simulink model "testrig_susp_knc"  (R2026a)
settings: Solver=ode23t  StopTime=309  MaxStep=0.05  AbsTol=1e-3  EnableMultiTasking=on
PostLoadFcn:
  | sm_car_load_vehicle_data('none','000');
  | Vehicle = sm_car_vehcfg_setPeopleOnOff(Vehicle,[0 0 0 0 0],'SuspA1');
  | set_param([bdroot '/Axle'],'AxNum','Front');
  | set_param([bdroot '/Axle/Visuals'],'popup_vis_point','Off');
  | 
  | Maneuver = MDatabase.KnC.Sedan_HambaLG;
  | Visual = sm_car_param_visual('default');
undefined symbols (not defined in the file or in its folder): Axle1D, AxleIn, Init, RaceFix, RaceSpin, X, Y, Z
libraries: sm_lib x9, sm_car_testrig_utilities_lib x6, fl_lib x4, Damper_Element x2, Spring_Element x2, nesl_utility x1, Damper_Control x1, Suspension x1, World_Config_Utilities x1
CloseFcn:
  | clear simlog_sm_car_testrig_quarter_car
  | clear logsout_sm_car_testrig_quarter_car
Description:
  | Half Car Testrig, Pullrod
  | 
  | Copyright 2021-2026 The MathWorks, Inc.
settings Model: Creator=smiller  LastModifiedBy=smiller
settings DataIOCC: SignalLoggingName=logsout_sm_car_testrig_quarter_car
settings SimscapeCC: SimscapeNominalValues="[{\"value\":\"1\",\"unit\":\"A\"},{\"value\":\"1\",\"unit\":\"bar\"},{\"value\":\"1\",\"unit\":\"cm^2\"},{\"value\":\"1\",\"unit\":\"cm^3/s\"},{\"value\":\"1\",\"unit\":\"kJ/kg\"},{\"value\":\"1\",\"unit\":\"kW\"},{\"value\":\"1\",\"unit\":\"l\"},{\"value\":\"1\",\"unit\":\"N\"},{\"value\":\"1\",\"unit\":\"N*m\"},{\"value\":\"1\",\"unit\":\"V\"}]"  SimscapeLogSimulationStatistics=on  SimscapeLogName=simlog_sm_car_testrig_quarter_car  SimscapeLogLimitData=off  SimscapeOperatingPoint=op
settings DiagnosticsConfigSet: SimMechanicsUnconnectedFramePorts=none  SimMechanicsConflictingReferenceFrames=none
settings ExplorerConfigSet: InternalSimMechanicsExplorerSettings="<ExplorerConfiguration><canonicalview>default</canonicalview><AnimationSetting><BasePlaybackSpeed>1.0</BasePlaybackSpeed><PlaybackSpeedFactor>16.0</PlaybackSpeedFactor></AnimationSetting><TilePanel><TileInfo><Tiles Columns=\"1\" Count=\"1\" Rows=\"1\"><Column Weight=\"1\"/><Row Weight=\"1\"/><Tile Height=\"1\" Width=\"1\" X=\"0\" Y=\"0\"/></Tiles></TileInfo><SceneInfo><SceneViewer><BGColor><R>1</R><G>1</G><B>1</B></BGColor><Camera><DoPerspective>off</DoPerspective><Position><X>0.571928528858414942</X><Y>-0.579111562749420217</Y><Z>0.83606068842340453</Z></Position><Center><X>-0.00542174033121090027</X><Y>-0.00176129355979437463</Y><Z>0.258710419233778688</Z></Center><Up><X>-0.408248290463863073</X><Y>0.408248290463863073</Y><Z>0.816496580927726145</Z></Up><ViewLimDist>1</ViewLimDist><YLim>0.718679582981457732</YLim><XLim>0.891323281686500546</XLim></Camera></SceneViewer></SceneInfo></TilePanel><MechEditorPanel><Cameras/><GfxPanelCameraMap/><VideoCreator><PlaybackSpeedRatio>1.0</PlaybackSpeedRatio><FrameRate>30</FrameRate><VideoFormat>Motion JPEG AVI</VideoFormat><FrameSize>auto</FrameSize></VideoCreator></MechEditorPanel></ExplorerConfiguration>"

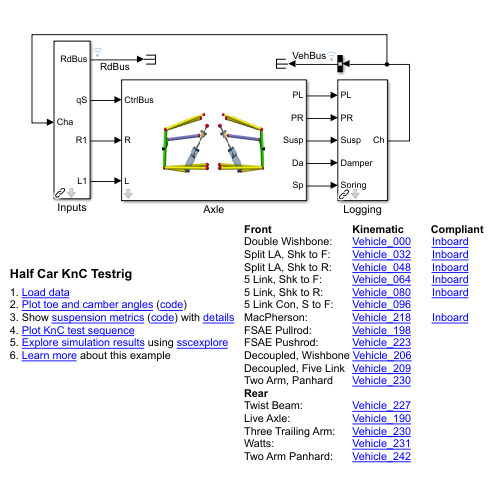
[thumbnail: Simulink's stored preview of the top-level diagram]
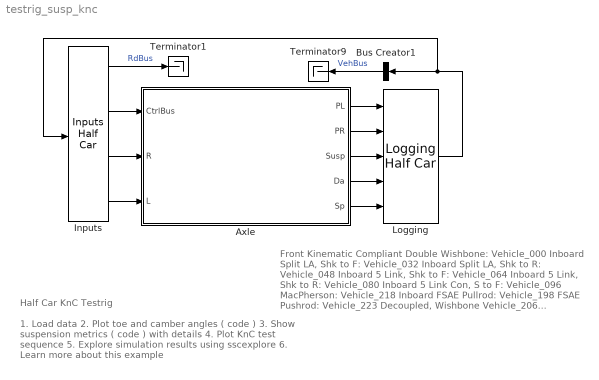
== system testrig_susp_knc ==
  note: Half Car KnC Testrig
  note: 1. Load data
      | 2. Plot toe and camber angles ( code )
      | 3. Show suspension metrics ( code ) with details
      | 4. Plot KnC test sequence
      | 5. Explore simulation results using sscexplore
      | 6. Learn more about this example
  note: Front Kinematic Compliant
      | Double Wishbone: Vehicle_000 Inboard
      | Split LA, Shk to F: Vehicle_032 Inboard
      | Split LA, Shk to R: Vehicle_048 Inboard
      | 5 Link, Shk to F: Vehicle_064 Inboard
      | 5 Link, Shk to R: Vehicle_080 Inboard
      | 5 Link Con, S to F: Vehicle_096
      | MacPherson: Vehicle_218 Inboard
      | FSAE Pullrod: Vehicle_198
      | FSAE Pushrod: Vehicle_223
      | Decoupled, Wishbone Vehicle_206
      | Decoupled, Five Link Vehicle_209
      | Two Arm, Panhard Vehicle_230
      | Rear
      | Twist Beam: Vehicle_227
      | Live Axle: Vehicle_190
      | Three Trailing Arm: Vehicle_230
      | Watts: Vehicle_231
      | Two Arm Panhard: Vehicle_242
  Axle : Subsystem  mask{AxNum=Front, Vehicle=Vehicle, popup_damper_control=None}
      mask prompts: AxNum "Axle"; Vehicle "Vehicle (structure)"; popup_damper_control "Damper Control"
      mask init:
      | curblk = gcb;
      | 
      | sWctrSet = sm_car_get_sWheelCentre(Vehicle);
      | sWCtr     = sWctrSet(AxNum,:);
      | 
      | tire_radii = sm_car_get_TireRadius(Vehicle);
      | tire_radius = tire_radii(AxNum);
      | 
      | if(AxNum==1)
      |     axleField = 'Axle1';
      |     suspField = 'SuspA1';
      |     tireField = 'TireA1';
      | else
      |     axleField = 'Axle2';
      |     suspField = 'SuspA2';
      |     tireField = 'TireA2';
      | end
      | 
      | if(strcmp(Vehicle.Chassis.(suspField).class.Value,'Decoupled'))
      |     springLparam = Vehicle.Chassis.Spring.(axleField).Heave;
      |     springLclass = Vehicle.Chassis.Spring.(axleField).Heave.class.Value;
      |     springRparam = Vehicle.Chassis.Spring.(axleField).Roll;
      |     springRclass = Vehicle.Chassis.Spring.(axleField).Roll.class.Value;
      |     damperLparam = Vehicle.Chassis.Damper.(axleField).Heave;
      |     damperLclass = Vehicle.Chassis.Damper.(axleField).Heave.class.Value;
      |     damperRparam = Vehicle.Chassis.Damper.(axleField).Roll;
      |     damperRclass = Vehicle.Chassis.Damper.(axleField).Roll.class.Value;
      | elseif(strcmp(Vehicle.Chassis.(suspField).class.Value,'LUT') || ...
      |         strcmp(Vehicle.Chassis.(suspField).class.Value,'Simple') )
      |     springLparam = 0;
      |     springLclass = 'No_Spring';
      |     springRparam = 0;
      |     springRclass = 'No_Spring';
      |     damperLparam = 0;
      |     damperLclass = 'None';
      |     damperRparam = 0;
      |     damperRclass = 'None';
      | elseif(strcmp(Vehicle.Chassis.(suspField).class.Value,'AxleTA2PR') || ...
      |         strcmp(Vehicle.Chassis.(suspField).class.Value,'AxleTA2PRNoSteer') )
      |     springLparam          = Vehicle.Chassis.Spring.(axleField);
      |     springLparam.sTop     = Vehicle.Chassis.Spring.(axleField).sTopL;
      |     springLparam.sBottom  = Vehicle.Chassis.Spring.(axleField).sBottomL;
      |     springLparam.xPreload = Vehicle.Chassis.Spring.(axleField).xPreloadL;
      |     springLparam.fPreload = Vehicle.Chassis.Spring.(axleField).fPreloadL;
      |     springLclass   = strrep(Vehicle.Chassis.Spring.(axleField).class.Value,'Asymmetric','');
      | 
      |     springRparam          = Vehicle.Chassis.Spring.(axleField);
      |     springRparam.sTop     = Vehicle.Chassis.Spring.(axleField).sTopR;
      |     springRparam.sBottom  = Vehicle.Chassis.Spring.(axleField).sBottomR;
      |     springRparam.xPreload = Vehicle.Chassis.Spring.(axleField).xPreloadR;
      |     springRparam.fPreload = Vehicle.Chassis.Spring.(axleField).fPreloadR;
      |     springRclass  =  strrep(Vehicle.Chassis.Spring.(axleField).class.Value,'Asymmetric','');
      |     
      |     damperLparam                 = Vehicle.Chassis.Damper.(axleField);
      |     damperLparam.Damping.sTop    = Vehicle.Chassis.Damper.(axleField).Damping.sTopL;
      |     damperLparam.Damping.sBottom = Vehicle.Chassis.Damper.(axleField).Damping.sBottomL;
      |     damperLclass          = strrep(Vehicle.Chassis.Damper.(axleField).class.Value,'Asymmetric','');
      | 
      |     damperRparam                 = Vehicle.Chassis.Damper.(axleField);
      |     damperRparam.Damping.sTop    = Vehicle.Chassis.Damper.(axleField).Damping.sTopR;
      |     damperRparam.Damping.sBottom = Vehicle.Chassis.Damper.(axleField).Damping.sBottomR;
      |     damperRclass          = strrep(Vehicle.Chassis.Damper.(axleField).class.Value,'Asymmetric','');
      | 
      | else
      |     springLparam = Vehicle.Chassis.Spring.(axleField);
      |     springLclass = Vehicle.Chassis.Spring.(axleField).class.Value;
      |     springRparam = Vehicle.Chassis.Spring.(axleField);
      |     springRclass = Vehicle.Chassis.Spring.(axleField).class.Value;
      |     damperLparam = Vehicle.Chassis.Damper.(axleField);
      |     damperLclass = Vehicle.Chassis.Damper.(axleField).class.Value;
      |     damperRparam = Vehicle.Chassis.Damper.(axleField);
      |     damperRclass = Vehicle.Chassis.Damper.(axleField).class.Value;
      | end
      mask TypeOptions AxNum: Front | Rear
      mask TypeOptions popup_damper_control: Damper Control /popup_damper_control
      mask Display:
      | curblk = gcb;
      | activeVar  = get_param([curblk '/Suspension'],'activevariant');
      | varChoices = get_param([curblk '/Suspension'],'VariantChoices');
      | 
      | varInd = find(strcmp(activeVar,{varChoices(:).Name}));
      | 
      | ActiveVarCmd = get_param(varChoices(varInd).BlockName,'MaskDisplay');
      | eval(ActiveVarCmd);
  Bus Creator1 : BusCreator  Inputs=1
  Inputs : sm_car_testrig_utilities_lib/Inputs Half Car  popup_steering_input=On
  Logging : sm_car_testrig_utilities_lib/Logging Half Car
  Terminator1 : Terminator
  Terminator9 : Terminator
  wires:
  Bus Creator1/1 -> Terminator9/1  "VehBus"
  Logging/1 -> Inputs/1, Bus Creator1/1
  Inputs/1 -> Terminator1/1  "RdBus"
  Inputs/3 -> Axle/2(R)
  Inputs/4 -> Axle/3(L)
  Inputs/2 -> Axle/1("CtrlBus ")
  Axle/1(PL) -> Logging/1
  Axle/2(PR) -> Logging/2
  Axle/3(Susp) -> Logging/3
  Axle/4(" Da") -> Logging/4
  Axle/5(" Sp") -> Logging/5

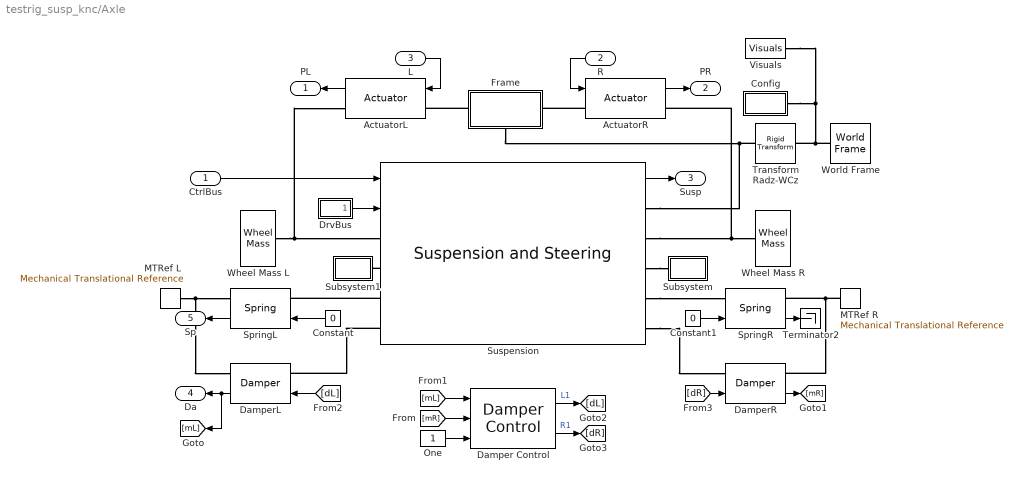
== system testrig_susp_knc/Axle ==
  "CtrlBus " : Inport
  R : Inport  Port=2
  L : Inport  Port=3
  ActuatorL : sm_car_testrig_utilities_lib/Actuator  tire_rad=tire_radius  xCPOffset=Maneuver.xCPOffset
  ActuatorR : sm_car_testrig_utilities_lib/Actuator  tire_rad=tire_radius  xCPOffset=Maneuver.xCPOffset
  Config : Subsystem
  Constant : Constant  Value=0
  Constant1 : Constant  Value=0
  "Damper Control " : Damper_Control/Damper Control   VariantControl=Choice  LabelModeActiveChoice=None  popup_damper_control=None  ControlDamper=Control.Damper.Axle1
      settings: AttributesFormatString=%<popup_damper_control>
  DamperL : Damper_Element/Damper  VariantControl=Variant1  LabelModeActiveChoice=Linear  Damper=damperLparam  VariantLabel=damperLclass
      settings: AttributesFormatString=%<ActiveVariant>
  DamperR : Damper_Element/Damper  VariantControl=Variant1  LabelModeActiveChoice=Linear  Damper=damperRparam  VariantLabel=damperRclass
      settings: AttributesFormatString=%<ActiveVariant>
  DrvBus : Subsystem
  Frame : Subsystem  mask{sWctr=sWCtr}
      mask prompts: sWctr "HP Wheel Center [x y z] (m)"
      settings: PortSchema="{\"entries\":[{\"content\":{\"sides\":[{\"content\":{\"connectorIds\":[\"LConn1\"]},\"type\":\"ConnectorPlacement.EquallySpacedRectSide\",\"uuid\":\"6bafd3c1-bcc7-4e93-aea7-1b45691869cb\"},{\"content\":{\"connectorIds\":[\"RConn1\"],\"side\":\"RIGHT\"},\"type\":\"ConnectorPlacement.EquallySpacedRectSide\",\"uuid\":\"8302b8de-ad89-4cb7-8500-2e46ba409587\"},{\"content\":{\"connectorIds\":[],\"side\":\"TOP\"},\"type\":\"ConnectorPlacement.EquallySpacedRectSide\",\"uuid\":\"64bfca4e-c32f-4ac3-9207-4b63dfa53628\"},{\"content\":{\"connectorIds\":[\"RConn2\"],\"side\":\"BOTTOM\"},\"type\":\"ConnectorPlacement.EquallySpacedRectSide\",\"uuid\":\"4259e7bb-430d-411d-8823-9d547be42692\"}]},\"type\":\"ConnectorPlacement.EquallySpacedConnector\",\"uuid\":\"5df32ab5-9c2e-4acb-a8ad-c01b5f56a7cb\"}],\"packageUris\":[\"http://schema.mathworks.com/mf0/Connector/R2020b\"],\"version\":\"1.0\"}"
  MTRef L : fl_lib/Mechanical/Translational Elements/Mechanical Translational Reference
  MTRef R : fl_lib/Mechanical/Translational Elements/Mechanical Translational Reference
  One : Constant  OutDataTypeStr=Inherit: Inherit via back propagation
  SpringL : Spring_Element/Spring  VariantControl=Variant1  LabelModeActiveChoice=Linear  Spring=springLparam  VariantLabel=springLclass
      settings: AttributesFormatString=%<ActiveVariant>
  SpringR : Spring_Element/Spring  VariantControl=Variant1  LabelModeActiveChoice=Linear  Spring=springRparam  VariantLabel=springRclass
      settings: AttributesFormatString=%<ActiveVariant>
  Subsystem : Subsystem
  Subsystem1 : Subsystem
  Suspension : Suspension/Suspension and Steering  VariantControl=Variant1  LabelModeActiveChoice=Linkage  Susp=Vehicle.Chassis.(suspField)  Init=Init.(axleField)  VariantLabel=Vehicle.Chassis.(suspField).class.Value
      settings: AttributesFormatString=%<LabelModeActiveChoice>
  Terminator2 : Terminator
  Transform Radz-WCz : sm_lib/Frames and Transforms/Rigid Transform  RotationMethod=None  FollAlignAxisA=+X  BaseAlignAxisA=+Y  FollAlignAxisB=+Y  BaseAlignAxisB=+Z  RotationStandardAxis=+Z  RotationAngle=0.0  RotationAngleUnits=deg  RotationArbitraryAxis=[0 0 1]  RotationSequenceAxes=FollowerAxes  RotationSequence=XYX  RotationSequenceAngles=[0 0 0]  RotationSequenceAnglesUnits=deg  RotationMatrix=[1 0 0; 0 1 0; 0 0 1]  Quaternion=[1 0 0 0]  TranslationMethod=StandardAxis  TranslationCartesianOffset=[0 0 0]  TranslationCartesianOffsetUnits=m  TranslationStandardAxis=+Z  TranslationStandardOffset=+(tire_radius-sWCtr(3))  TranslationStandardOffsetUnits=m  TranslationROffset=0  TranslationROffsetUnits=m  TranslationThetaOffset=0  TranslationThetaOffsetUnits=deg  TranslationZOffset=0  TranslationZOffsetUnits=m
  Visuals : World_Config_Utilities/Visuals  VariantControl=Choice  LabelModeActiveChoice=Off  popup_vis_point=Off  time_vector=0  xyz_matrix=[0 0 0]  clr_vis=[0.0 1.0 0.8]  opc_vis=0.6  rad_vis=0.03
  Wheel Mass L : sm_car_testrig_utilities_lib/Wheel Mass  tire_param=Vehicle.Chassis.(tireField).tirFile.Value
  Wheel Mass R : sm_car_testrig_utilities_lib/Wheel Mass  tire_param=Vehicle.Chassis.(tireField).tirFile.Value
  World Frame : sm_lib/Frames and Transforms/World Frame
  PL : Outport
  PR : Outport  Port=2
  Susp : Outport  Port=3
  " Da" : Outport  Port=4
  " Sp" : Outport  Port=5
  wires:
  DamperL/1 -> [mL], " Da"/1
  "CtrlBus "/1 -> Suspension/1
  Constant1/1 -> SpringR/1
  DamperR/1 -> [mR]
  SpringL/1 -> " Sp"/1
  SpringR/1 -> Terminator2/1
  Constant/1 -> SpringL/1
  ActuatorL/1 -> PL/1
  DrvBus/1(Out1) -> Suspension/2
  Suspension/1 -> Susp/1
  R/1 -> ActuatorR/1
  L/1 -> ActuatorL/1
  ActuatorR/1 -> PR/1
  [mR] -> "Damper Control "/2
  [mL] -> "Damper Control "/1
  One/1 -> "Damper Control "/3
  "Damper Control "/1 -> [dL]  "L1"
  [dL] -> DamperL/1
  "Damper Control "/2 -> [dR]  "R1"
  [dR] -> DamperR/1
  connections:
  Suspension/RConn3 -- Subsystem/LConn1
  Suspension/RConn5 -- DamperR/LConn1
  Suspension/RConn1 -- Frame/RConn2 -- Transform Radz-WCz/RConn1
  Suspension/RConn2 -- ActuatorR/RConn1 -- Wheel Mass R/RConn1
  Suspension/LConn3 -- SpringL/LConn1
  Suspension/RConn4 -- SpringR/LConn1
  MTRef L/LConn1 -- SpringL/RConn1 -- DamperL/RConn1
  Wheel Mass L/RConn1 -- ActuatorL/RConn1 -- Suspension/LConn1
  Frame/LConn1 -- ActuatorL/LConn1
  MTRef R/LConn1 -- DamperR/RConn1 -- SpringR/RConn1
  ActuatorR/LConn1 -- Frame/RConn1
  Suspension/LConn4 -- DamperL/LConn1
  Suspension/LConn2 -- Subsystem1/LConn1
  Config/RConn1 -- Visuals/LConn1 -- World Frame/RConn1 -- Transform Radz-WCz/LConn1

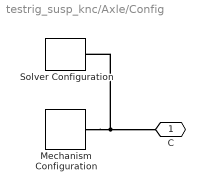
== system testrig_susp_knc/Axle/Config ==
  Mechanism Configuration : sm_lib/Utilities/Mechanism Configuration  UniformGravity=Constant  GravityVector=[0 0 -9.80665]  GravityVectorUnits=m/s^2  LinearizationDelta=0.001  JointModeTransitionNonlinearIterations=2
  Solver Configuration : nesl_utility/Solver Configuration  PhysicalDomain=network_engine_domain  SubClassName=solver  LeftPortType=input  RightPortType=generic  Tones=[]  Harmonics=[]  SimulateNoise=off  Profile=off  UseLocalSampling=off  EnableSwitchedLinearOptims=on  FrequencyDomain=off  UseCCode=off  RelTol=0.001  AbsTol=1e-06  MinStep=1e-09  ToWorkspace=off  RevertToSquareIcSolve=off  NumHomotopyIterations=100  PhasorMode=off  PhasorModeNumHarmonics=1  ConsistencySolver=NEWTON_FTOL  CanonicalOrdering=UNORDERED  OptimizeIntermediates=UNOPTIMIZED  IndexReductionMethod=DerivativeReplacement  DoDC=off  ResidualTolerance=1e-09  ConsistencyTolSource=GLOBAL  ConsistencyAbsTol=0.001  ConsistencyRelTol=0.001  ConsistencyTolFactor=0.001  UseLocalSolver=off  LocalSolverChoice=NE_BACKWARD_EULER_ADVANCER  ResolveIndetEquations=on  FunctionEvalNumThread=1  LocalSolverSampleTime=0.001  DoFixedCost=off  MaxNonlinIter=3  MaxModeIter=2  ComputeImpulses=off  ImpulseIterations=2  LinearAlgebra=Sparse  LinearAlgebraNumThread=0  EquationFormulation=NE_TIME_EF  DelaysMemoryBudget=1024  AutomaticFiltering=on  FilteringTimeConstant=0.001  PartitionStorageMethod=AS_NEEDED  PartitionMemoryBudget=1024  PartitionMethod=FAST  MultibodyUseLocalSolver=off  MultibodyLocalSolverChoice=ODE1  MultibodyLocalSolverSampleTime=0.001
  C : PMIOPort  Side=Right
  connections:
  Mechanism Configuration/RConn1 -- Solver Configuration/RConn1 -- C/RConn1

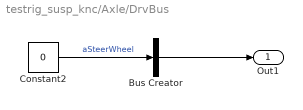
== system testrig_susp_knc/Axle/DrvBus ==
  Bus Creator : BusCreator  Inputs=1
  Constant2 : Constant  Value=0
  Out1 : Outport
  wires:
  Constant2/1 -> Bus Creator/1  "aSteerWheel"
  Bus Creator/1 -> Out1/1

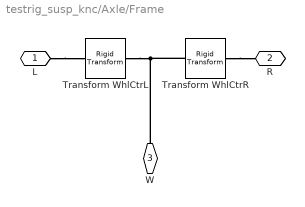
== system testrig_susp_knc/Axle/Frame ==
  Transform WhlCtrL : sm_lib/Frames and Transforms/Rigid Transform  RotationMethod=None  FollAlignAxisA=+X  BaseAlignAxisA=+Y  FollAlignAxisB=+Y  BaseAlignAxisB=+Z  RotationStandardAxis=+Z  RotationAngle=0.0  RotationAngleUnits=deg  RotationArbitraryAxis=[0 0 1]  RotationSequenceAxes=FollowerAxes  RotationSequence=XYX  RotationSequenceAngles=[0 0 0]  RotationSequenceAnglesUnits=deg  RotationMatrix=[1 0 0; 0 1 0; 0 0 1]  Quaternion=[1 0 0 0]  TranslationMethod=Cartesian  TranslationCartesianOffset=sWctr  TranslationCartesianOffsetUnits=m  TranslationStandardAxis=+Z  TranslationStandardOffset=0  TranslationStandardOffsetUnits=m  TranslationROffset=0  TranslationROffsetUnits=m  TranslationThetaOffset=0  TranslationThetaOffsetUnits=deg  TranslationZOffset=0  TranslationZOffsetUnits=m
  Transform WhlCtrR : sm_lib/Frames and Transforms/Rigid Transform  RotationMethod=None  FollAlignAxisA=+X  BaseAlignAxisA=+Y  FollAlignAxisB=+Y  BaseAlignAxisB=+Z  RotationStandardAxis=+Z  RotationAngle=0.0  RotationAngleUnits=deg  RotationArbitraryAxis=[0 0 1]  RotationSequenceAxes=FollowerAxes  RotationSequence=XYX  RotationSequenceAngles=[0 0 0]  RotationSequenceAnglesUnits=deg  RotationMatrix=[1 0 0; 0 1 0; 0 0 1]  Quaternion=[1 0 0 0]  TranslationMethod=Cartesian  TranslationCartesianOffset=sWctr.*[1 -1 1]  TranslationCartesianOffsetUnits=m  TranslationStandardAxis=+Z  TranslationStandardOffset=0  TranslationStandardOffsetUnits=m  TranslationROffset=0  TranslationROffsetUnits=m  TranslationThetaOffset=0  TranslationThetaOffsetUnits=deg  TranslationZOffset=0  TranslationZOffsetUnits=m
  L : PMIOPort  Side=Left
  R : PMIOPort  Port=2  Side=Right
  W : PMIOPort  Port=3  Side=Right
  connections:
  Transform WhlCtrR/LConn1 -- Transform WhlCtrL/LConn1 -- W/RConn1
  L/RConn1 -- Transform WhlCtrL/RConn1
  Transform WhlCtrR/RConn1 -- R/RConn1

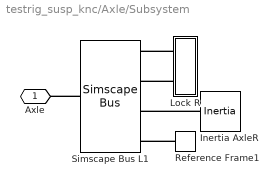
== system testrig_susp_knc/Axle/Subsystem ==
  Inertia AxleR : fl_lib/Mechanical/Rotational Elements/Inertia  inertia=0.01 kg*m^2  num_ports=foundation.enum.numPorts2.one  w_specify=on  w_priority=None  w=0 rad/s  w_nominal_specify=off  w_nominal_value=1  w_nominal_unit=rad/s  t_specify=off  t_priority=None  t=0 N*m  t_nominal_specify=off  t_nominal_value=1  t_nominal_unit=N*m
  Lock R : Subsystem
  Reference Frame1 : sm_lib/Frames and Transforms/Reference Frame
  Simscape Bus L1 : SimscapeBus  HierarchyStrings=RaceSpin;RaceFix;Axle1D;AxleIn
  Axle : PMIOPort  Side=Left
  connections:
  Lock R/LConn2 -- Simscape Bus L1/LConn2
  Reference Frame1/RConn1 -- Simscape Bus L1/LConn4
  Lock R/LConn1 -- Simscape Bus L1/LConn1
  Inertia AxleR/LConn1 -- Simscape Bus L1/LConn3
  Simscape Bus L1/RConn1 -- Axle/RConn1

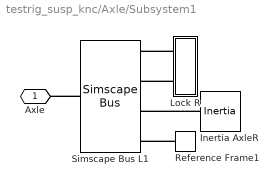
== system testrig_susp_knc/Axle/Subsystem1 ==
  Inertia AxleR : fl_lib/Mechanical/Rotational Elements/Inertia  inertia=0.01 kg*m^2  num_ports=foundation.enum.numPorts2.one  w_specify=on  w_priority=None  w=0 rad/s  w_nominal_specify=off  w_nominal_value=1  w_nominal_unit=rad/s  t_specify=off  t_priority=None  t=0 N*m  t_nominal_specify=off  t_nominal_value=1  t_nominal_unit=N*m
  Lock R : Subsystem
  Reference Frame1 : sm_lib/Frames and Transforms/Reference Frame
  Simscape Bus L1 : SimscapeBus  HierarchyStrings=RaceSpin;RaceFix;Axle1D;AxleIn
  Axle : PMIOPort  Side=Left
  connections:
  Simscape Bus L1/RConn1 -- Axle/RConn1
  Inertia AxleR/LConn1 -- Simscape Bus L1/LConn3
  Lock R/LConn1 -- Simscape Bus L1/LConn1
  Reference Frame1/RConn1 -- Simscape Bus L1/LConn4
  Lock R/LConn2 -- Simscape Bus L1/LConn2

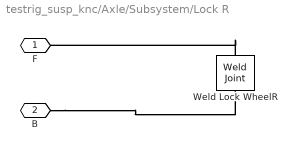
== system testrig_susp_knc/Axle/Subsystem/Lock R ==
  Weld Lock WheelR : sm_lib/Joints/Weld Joint  JointMode=Normal  CompositeWrenchDir=FollowerOnBase  CompositeWrenchFrame=BaseFrame  SenseConstraintForce=off  SenseConstraintTorque=off  SenseTotalForce=off  SenseTotalTorque=off
  F : PMIOPort  Side=Left
  B : PMIOPort  Port=2  Side=Left
  connections:
  Weld Lock WheelR/RConn1 -- F/RConn1
  B/RConn1 -- Weld Lock WheelR/LConn1

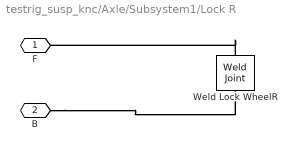
== system testrig_susp_knc/Axle/Subsystem1/Lock R ==
  Weld Lock WheelR : sm_lib/Joints/Weld Joint  JointMode=Normal  CompositeWrenchDir=FollowerOnBase  CompositeWrenchFrame=BaseFrame  SenseConstraintForce=off  SenseConstraintTorque=off  SenseTotalForce=off  SenseTotalTorque=off
  F : PMIOPort  Side=Left
  B : PMIOPort  Port=2  Side=Left
  connections:
  B/RConn1 -- Weld Lock WheelR/LConn1
  Weld Lock WheelR/RConn1 -- F/RConn1
